simulink model "final_project"  (R2026a)
settings: Solver=FixedStepDiscrete  StopTime=10  FixedStep=0.004
undefined symbols (not defined in the file): dspblkCoreblockFVToolHelper, gcbh
libraries: simulink x3, dspmlti4 x2, dspfdesign x2, dspstat3 x2, dspsigops x1
settings Model: Creator=Acer  LastModifiedBy=Acer

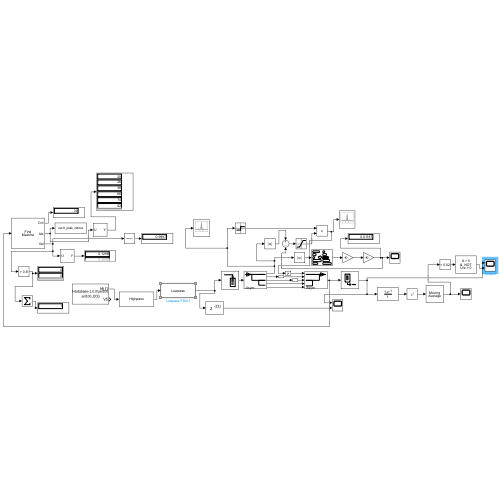
[thumbnail: Simulink's stored preview of the top-level diagram]
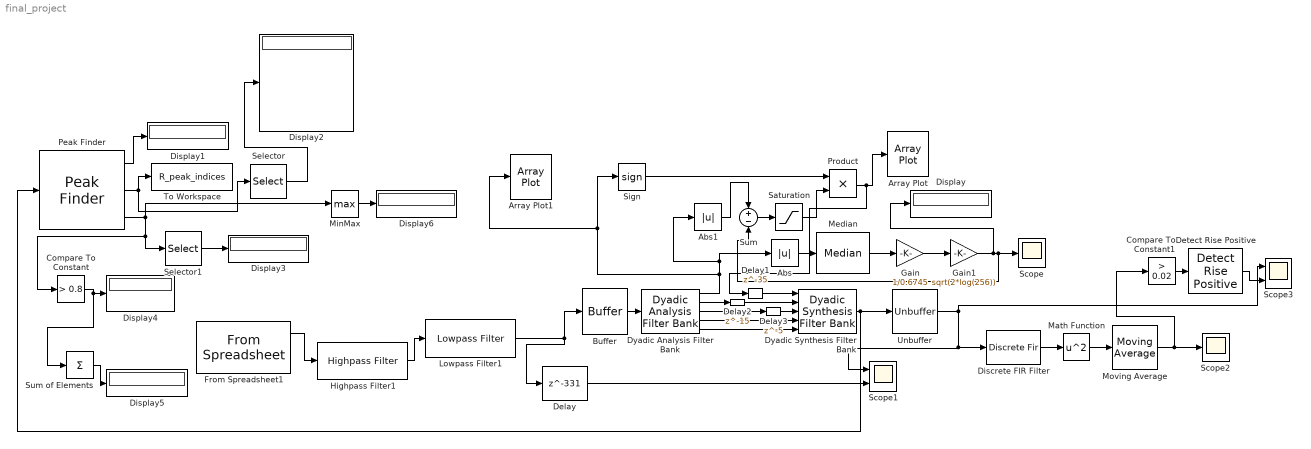
== system final_project ==
  Abs : Abs  SaturateOnIntegerOverflow=off
  Abs1 : Abs  SaturateOnIntegerOverflow=off
  Array Plot : ArrayPlot  WindowPosition=[-106.000000,174.000000,800.000000,500.000000,]  ScopeFrameLocation=window  YLimits=[-0.0739 0.0646]
  Array Plot1 : ArrayPlot  WindowPosition=[696.000000,164.000000,800.000000,500.000000,]  ScopeFrameLocation=window  YLimits=[-0.0872 0.0779]
  Buffer : Buffer  N=256  OutputFrames=off
  Compare To Constant : simulink/Logic and Bit Operations/Compare To Constant  relop=>  const=0.8  OutDataTypeStr=boolean
  Compare To Constant1 : simulink/Logic and Bit Operations/Compare To Constant  relop=>  const=0.02  OutDataTypeStr=boolean
  Delay : Delay  DelayLength=331
  Delay1 : Delay  DelayLength=35  InputProcessing=Columns as channels (frame based)
  Delay2 : Delay  DelayLength=15  InputProcessing=Columns as channels (frame based)
  Delay3 : Delay  DelayLength=5  InputProcessing=Columns as channels (frame based)
  Detect Rise Positive : simulink/Logic and Bit Operations/Detect Rise Positive  vinit=0  OutDataTypeStr=boolean
  Discrete FIR Filter : DiscreteFir  LoadFcn=dspblkCoreblockFVToolHelper(gcbh,'load');  Coefficients=[1 -1]
      settings: CopyFcn=dspblkCoreblockFVToolHelper(gcbh,'copy');  DeleteFcn=dspblkCoreblockFVToolHelper(gcbh,'close');  ModelCloseFcn=dspblkCoreblockFVToolHelper(gcbh,'close');  PreSaveFcn=dspblkCoreblockFVToolHelper(gcbh,'presave');  PostSaveFcn=dspblkCoreblockFVToolHelper(gcbh,'postsave');  CloseFcn=dspblkCoreblockFVToolHelper(gcbh,'close');
  Display{,1..6} (7 alike) : Display
  Dyadic Analysis Filter Bank : dspmlti4/Dyadic Analysis Filter Bank  Wname=User-defined  OrdRec_ordDec=[1 / 1]  Order=2  LPF="[0.0352   -0.0854   -0.1350   0.4599   0.8069   0.3327]"  HPF="[-0.3327    0.8069   -0.4599   -0.1350    0.0854    0.0352]"  NumLevels=4  tree=Asymmetric  Output=Multiple ports  OutputFrames=off
  Dyadic Synthesis Filter Bank : dspmlti4/Dyadic Synthesis Filter Bank  Wname=User-defined  OrdRec_ordDec=[1 / 1]  Order=2  LPF="[0.3327    0.8069    0.4599   -0.1350   -0.0854    0.0352]"  HPF="[0.0352    0.0854   -0.1350   -0.4599    0.8069   -0.3327]"  NumLevels=4  tree=Asymmetric  Input=Multiple ports  OutputFrames=off
  From Spreadsheet1 : FromSpreadsheet  FileName=D:\dsp\qt-database-1.0.0\sel100_ECG.csv  SheetName=sel100_ECG  SampleTime=0.004
  Gain : Gain  Gain=1/0.6745
  Gain1 : Gain  Gain=sqrt(2*log(256))
  Highpass Filter1 : dspfdesign/Highpass Filter  FilterType=IIR  DesignForMinimumOrder=on  FilterOrder=50  StopbandFrequency=0.2  PassbandFrequency=0.5  StopbandAttenuation=40  PassbandRipple=0.1  SampleRateMode=Specify on dialog  SampleRate=250  SimulateUsing=Interpreted execution  roundingMode=Floor  coeffsDataTypeStr=fixdt(1,16)
  Lowpass Filter1 : dspfdesign/Lowpass Filter  FilterType=IIR  DesignForMinimumOrder=on  FilterOrder=50  PassbandFrequency=40  StopbandFrequency=50  PassbandRipple=0.5  StopbandAttenuation=40  SampleRateMode=Specify on dialog  SampleRate=250  SimulateUsing=Interpreted execution  roundingMode=Floor  coeffsDataTypeStr=fixdt(1,16)
  Math Function : Math  Operator=square
  Median : dspstat3/Median  sortAlg=Quick sort  directionMode=Entire input  dimension=1  roundingMode=Floor  overflowMode=off  accumDataTypeStr=Inherit: Same as product output  accumLastDataTypeStr=Inherit: Same as product output  outputDataTypeStr=Inherit: Same as accumulator  outputMin=[]  outputMax=[]  outputLastDataTypeStr=Inherit: Same as accumulator
      settings: allowOverrides=off
  MinMax : MinMax  Function=max
  Moving Average : dspstat3/Moving Average  Method=Sliding window  ForgettingFactorPort=off  SpecifyWindowLength=on  WindowLengthSource=Property  MaxWindowLength=20  WindowLength=30  OverlapLength=29  AllowArbitraryInputLength=off  ForgettingFactor=0.9  SimulateUsing=Interpreted execution
  Peak Finder : dspsigops/Peak Finder  polarity=Maxima  indexBase=One  outputIdx=on  outputVal=on  maxPeaks=128  NoiseDistinguish=off  thresh=0  roundingMode=Floor  overflowMode=off
      settings: allowOverrides=off
  Product : Product
  Saturation : Saturate  UpperLimit=inf  LowerLimit=0
  Scope : Scope
      settings: ActiveDisplayYMinimum=-1  ActiveDisplayYMaximum=1
  Scope1 : Scope  NumInputPorts=2
      settings: ActiveDisplayYMinimum=-2.7374649427487565  ActiveDisplayYMaximum=5.7888190361821037
  Scope2 : Scope
      settings: ActiveDisplayYMinimum=-0.027065916417386742  ActiveDisplayYMaximum=0.24359324775648075  DataLoggingVariableName=ScopeData2
  Scope3 : Scope  NumInputPorts=2
      settings: ActiveDisplayYMinimum=-2.6519501888127568  ActiveDisplayYMaximum=5.7881439619046642  DataLoggingVariableName=ScopeData3
  Selector : Selector  InputPortWidth=128  IndexOptions=Index vector (dialog)  Indices=1:10  OutputSizes=1
  Selector1 : Selector  InputPortWidth=128  IndexOptions=Index vector (dialog)  Indices=1:10  OutputSizes=1
  Sign : Signum
  Sum : Sum  Inputs=+-
  Sum of Elements : Sum  Inputs=+
  To Workspace : ToWorkspace  VariableName=R_peak_indices  SaveFormat=Timeseries  SampleTime=-1
  Unbuffer : Unbuffer
  wires:
  Saturation/1 -> Product/2
  From Spreadsheet1/1 -> Highpass Filter1/1
  Dyadic Analysis Filter Bank/4 -> Dyadic Synthesis Filter Bank/4
  Product/1 -> Delay1/1, Array Plot/1
  Delay1/1 -> Dyadic Synthesis Filter Bank/1
  Highpass Filter1/1 -> Lowpass Filter1/1
  Gain1/1 -> Display/1, Sum/2, Scope/1
  Sum/1 -> Saturation/1
  Dyadic Analysis Filter Bank/2 -> Delay2/1
  Median/1 -> Gain/1
  Dyadic Analysis Filter Bank/3 -> Delay3/1
  Gain/1 -> Gain1/1
  Sign/1 -> Product/1
  Buffer/1 -> Dyadic Analysis Filter Bank/1
  Delay2/1 -> Dyadic Synthesis Filter Bank/2
  Dyadic Analysis Filter Bank/5 -> Dyadic Synthesis Filter Bank/5
  Delay/1 -> Scope1/2
  Unbuffer/1 -> Discrete FIR Filter/1, Scope1/1, Scope3/1
  Abs1/1 -> Sum/1
  Abs/1 -> Median/1
  Dyadic Analysis Filter Bank/1 -> Array Plot1/1, Sign/1, Abs1/1, Abs/1
  Lowpass Filter1/1 -> Buffer/1, Delay/1
  Delay3/1 -> Dyadic Synthesis Filter Bank/3
  Dyadic Synthesis Filter Bank/1 -> Unbuffer/1, Peak Finder/1
  Peak Finder/1 -> Display1/1
  Peak Finder/2 -> Selector/1, To Workspace/1
  Selector/1 -> Display2/1
  Peak Finder/3 -> Compare To Constant/1, Selector1/1, MinMax/1
  Selector1/1 -> Display3/1
  Compare To Constant/1 -> Sum of Elements/1, Display4/1
  Sum of Elements/1 -> Display5/1
  MinMax/1 -> Display6/1
  Discrete FIR Filter/1 -> Math Function/1
  Math Function/1 -> Moving Average/1
  Moving Average/1 -> Compare To Constant1/1, Scope2/1
  Compare To Constant1/1 -> Detect Rise Positive/1
  Detect Rise Positive/1 -> Scope3/2
